simulink model "Rate_Limit_Test"  (R2023b)
settings: Solver=VariableStepAuto  StartTime=0.0  StopTime=50  RelTol=1e-3
libraries: simulink x1, simulink_need_slupdate x1
settings Model: Creator=FIRSTMentor  LastModifiedBy=FIRSTMentor

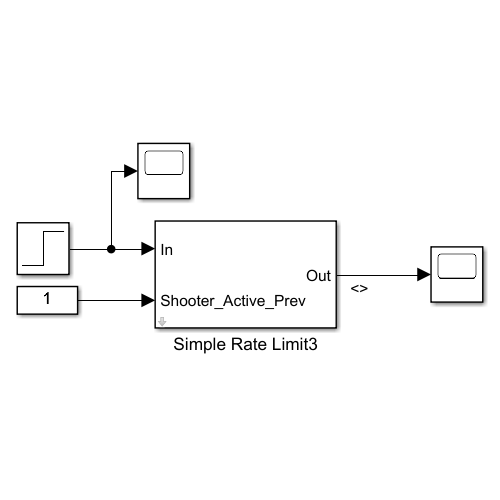
[thumbnail: Simulink's stored preview of the top-level diagram]
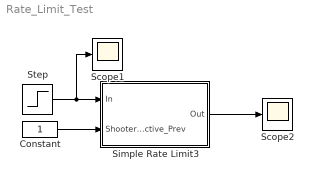
== system Rate_Limit_Test ==
  Constant : Constant
  Scope1 : Scope
  Scope2 : Scope
  Simple Rate Limit3 : Subsystem  mask{Rate_Limit_Inc=0.1, Rate_Limit_Dec=0.1}
  Step : Step  Time=0.1  SampleTime=0
  wires:
  Constant/1 -> Simple Rate Limit3/2(Shooter_Active_Prev)
  Simple Rate Limit3/1(Out) -> Scope2/1
  Step/1 -> Scope1/1, Simple Rate Limit3/1(In)

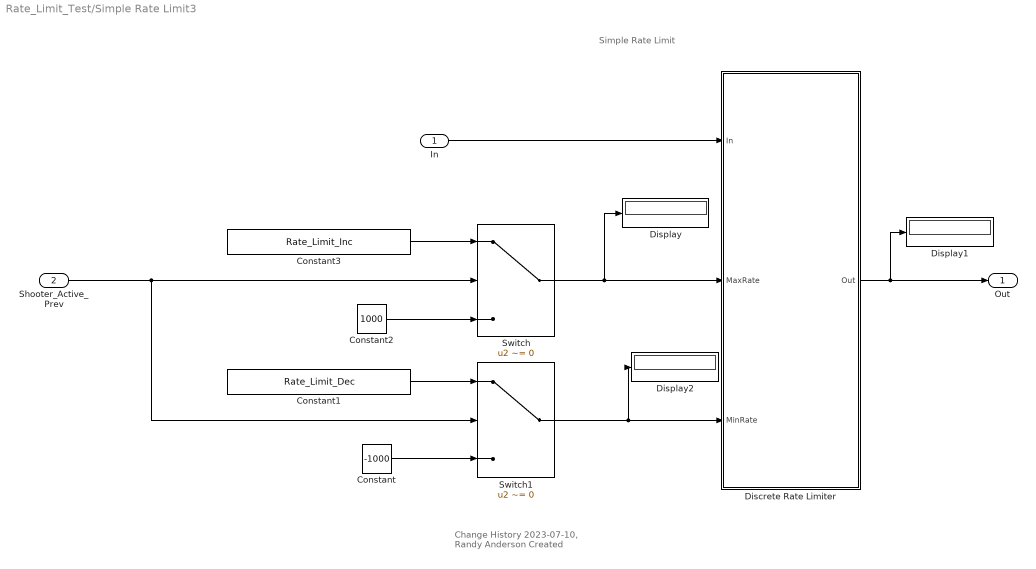
== system Rate_Limit_Test/Simple Rate Limit3 ==
  note: Simple Rate Limit
  note: Change History
      | 2023-07-10, Randy Anderson
      |     Created
  In : Inport
  Shooter_Active_Prev : Inport  Port=2
  Constant : Constant  Value=-1000
  Constant1 : Constant  Value=Rate_Limit_Dec
      settings: AttributesFormatString=%<OutDataTypeStr>
  Constant2 : Constant  Value=1000
  Constant3 : Constant  Value=Rate_Limit_Inc
      settings: AttributesFormatString=%<OutDataTypeStr>
  Discrete Rate Limiter : Subsystem
  Display : Display
  Display1 : Display
  Display2 : Display
  Switch : Switch  Criteria=u2 ~= 0  SaturateOnIntegerOverflow=off  InputSameDT=off
  Switch1 : Switch  Criteria=u2 ~= 0  SaturateOnIntegerOverflow=off  InputSameDT=off
  Out : Outport
  wires:
  In/1 -> Discrete Rate Limiter/1(In)
  Discrete Rate Limiter/1(Out) -> Display1/1, Out/1
  Constant3/1 -> Switch/1
  Shooter_Active_Prev/1 -> Switch/2, Switch1/2
  Constant1/1 -> Switch1/1
  Switch/1 -> Display/1, Discrete Rate Limiter/2(MaxRate)
  Switch1/1 -> Display2/1, Discrete Rate Limiter/3(MinRate)
  Constant/1 -> Switch1/3
  Constant2/1 -> Switch/3

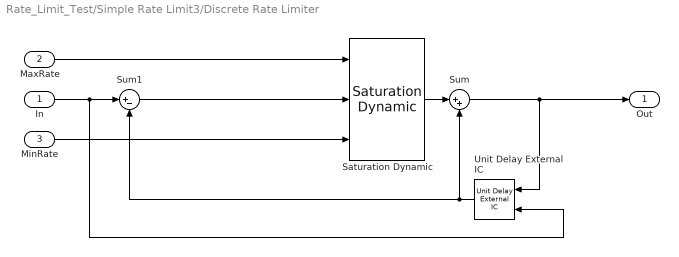
== system Rate_Limit_Test/Simple Rate Limit3/Discrete Rate Limiter ==
  In : Inport
  MaxRate : Inport  Port=2
  MinRate : Inport  Port=3
  Saturation Dynamic : simulink/Discontinuities/Saturation Dynamic  OutMin=[]  OutMax=[]  OutDataTypeStr=Inherit: Same as second input  OutDataType=fixdt(1, 16)  OutScaling=2^-10  DoSatur=off
  Sum : Sum  Inputs=|++  OutDataTypeStr=Inherit: Inherit via back propagation
  Sum1 : Sum  Inputs=|+-  OutDataTypeStr=Inherit: Inherit via back propagation  SaturateOnIntegerOverflow=on
  Unit Delay External IC : simulink_need_slupdate/Unit Delay External IC  tsamp=-1
  Out : Outport
  wires:
  Sum/1 -> Out/1, Unit Delay External IC/1
  MinRate/1 -> Saturation Dynamic/3
  MaxRate/1 -> Saturation Dynamic/1
  Saturation Dynamic/1 -> Sum/1
  Sum1/1 -> Saturation Dynamic/2
  Unit Delay External IC/1 -> Sum1/2, Sum/2
  In/1 -> Unit Delay External IC/2, Sum1/1
